simulink model "acc_carsim_interface"  (R2024a)
settings: Solver=FixedStepDiscrete  StartTime=0.0  StopTime=30  FixedStep=0.02  RelTol=1e-3
model workspace (MAT data in the model file):
  initialXo_m = 0
libraries: acc_control_lib x1
settings Model: Creator=26401  LastModifiedBy=26401

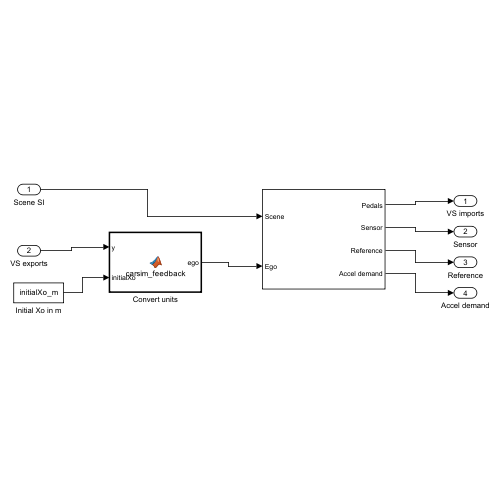
[thumbnail: Simulink's stored preview of the top-level diagram]
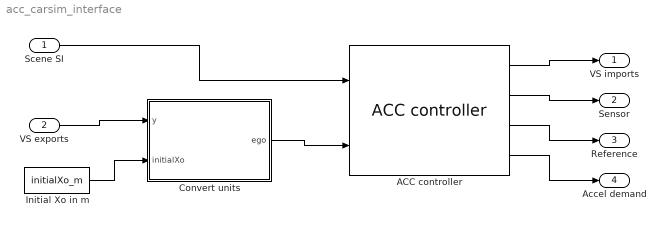
== system acc_carsim_interface ==
  Scene SI : Inport  PortDimensions=4  SampleTime=0.02
  VS exports : Inport  Port=2  PortDimensions=5  SampleTime=0.02
  ACC controller : acc_control_lib/ACC controller  SystemSampleTime=-1  VariantActivationTime=update diagram  AllowFlexibleInterface=on  Latency=0  AutoFrameSizeCalculation=off
  Convert units : MATLAB Function  TreatAsAtomicUnit=on
  Initial Xo in m : Constant  Value=initialXo_m
  VS imports : Outport
  Sensor : Outport  Port=2
  Reference : Outport  Port=3
  Accel demand : Outport  Port=4
  wires:
  ACC controller/1 -> VS imports/1
  ACC controller/2 -> Sensor/1
  ACC controller/3 -> Reference/1
  ACC controller/4 -> Accel demand/1
  Scene SI/1 -> ACC controller/1
  VS exports/1 -> Convert units/1(y)
  Initial Xo in m/1 -> Convert units/2(initialXo)
  Convert units/1(ego) -> ACC controller/2

== matlab function acc_carsim_interface/Convert units ==
  data: y input; ego output; initialXo input
function ego = carsim_feedback(y,initialXo)
% Paper Fig. 6 export order. Confirm native units in the active VS dataset.
% AV_Eng rpm, Rgear_TR ratio, Vx km/h, Xo m, Ax g.
% Straight road, fixed heading. Local s=0 is the initial ego front bumper.
ego = [y(4)-initialXo; y(3)/3.6; y(5)*9.80665; y(1); y(2)];
end
